simulink model "Shaddad_SensorModels"  (R2026b)
settings: Solver=VariableStepAuto
values from neighbouring files (symbols this model uses):
  D = zeros(nx, ny, 'uint8')    [sens_lidar2d_fast.m]
  P = (P + P.')/2    [sens_nav_ekf.m]
undefined symbols (not defined in the file or in its folder): sens_gnss_fixchain_prm, sens_lidar2d_fast_prm, Ts
libraries: sensorgpslib x3, uavsimlib x3, sharedutil x1
settings Model: Creator=aomar  LastModifiedBy=aomar

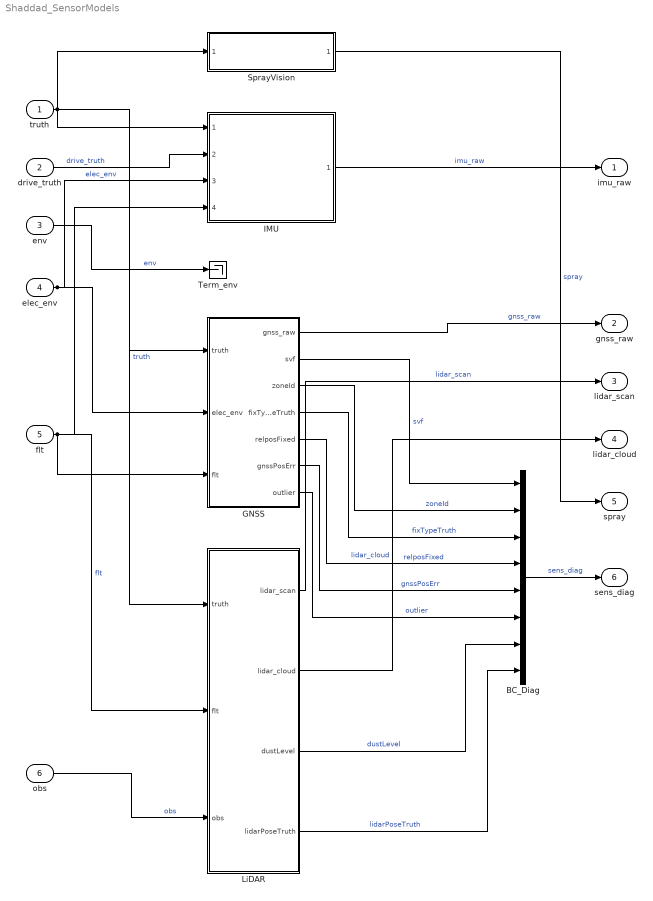
== system Shaddad_SensorModels ==
  truth : Inport  OutDataTypeStr=Bus: Bus_TruthState  SampleTime=Ts.base
  drive_truth : Inport  Port=2  OutDataTypeStr=Bus: Bus_DriveTruth  SampleTime=Ts.base
  env : Inport  Port=3  OutDataTypeStr=Bus: Bus_EnvState  SampleTime=Ts.hk
  elec_env : Inport  Port=4  OutDataTypeStr=Bus: Bus_ElecEnv  SampleTime=Ts.hk
  flt : Inport  Port=5  OutDataTypeStr=Bus: Bus_FaultInject  SampleTime=Ts.ctrl
  obs : Inport  Port=6  OutDataTypeStr=Bus: Bus_ObstaclesDyn  SampleTime=Ts.ctrl
  BC_Diag : BusCreator  Inputs=8  OutDataTypeStr=Bus: Bus_SensTruthDiag  NonVirtualBus=on
      settings: InheritFromInputs=off
  GNSS : Subsystem  Description=|
      | sens_gnss_model (T11, sensors spec 3.2). Ports: in 1 truth Bus_TruthState 0.001, 2 elec_env Bus_ElecEnv 0.1, 3 flt Bus_FaultInject 0.01; out 1 gnss_raw Bus_GnssRaw 0.1, 2 svf double, 3 zoneId uint8, 4 fixTypeTruth uint8, 5 relposFixed boolean, 6 gnssPosErr double[3] (reported - true antenna ENU), 7 outlier boolean (all 0.1).
      | p_a = pos_W + R_WB rAnt1, v_a = vel_W + R_WB (omega x rAnt1); Delay 8 x 0.01 s (latency) -> 0.1 s epochs; sky view = 2-D Lookup Tables P.world.gnssSvf (linear) / gnssZoneId (nearest) at the antenna xy (D59); fix chain MATLAB Function sens_gnss_fixchain (corrOK/corrAge from elec_env, gnss_outage / gnss_force_float from flt); three mspsensorlib/GPS (FIXED/FLOAT/SINGLE, position only: VelocityAccuracy 0) + Multiport Switch {4,5,1}; velocity v_a + N(0, sigVel(fix)^2) per axis (the GPS block's own velocity noise reads 1.2533 sigVel high along the track); outliers U(2,5) m; heading CW from N + N(0, 0.5 deg).
  IMU : Subsystem  ReferencedSubsystem=sens_imu_model
  LiDAR : Subsystem  Description=|
      | sens_lidar_model (T11, sensors spec 3.4). Ports: in 1 truth Bus_TruthState 0.001, 2 flt Bus_FaultInject 0.01, 3 obs Bus_ObstaclesDyn 0.01; out 1 lidar_scan Bus_LidarScanRaw 0.1, 2 lidar_cloud Bus_LidarCloudRaw 0.1, 3 dustLevel double 0.1, 4 lidarPoseTruth double[3] [x_E y_N psi] 0.1.
      | Variant Subsystem VC_LIDAR (update diagram): 1 FAST2D = MATLAB Function sens_lidar2d_fast (raster of P.world.obstacles at first call, film layer, dynamic obstacles from obs, dust, blackout), cloud = P.ic; 2 FULL3D = uavsimlib UAV Scenario Configuration (sens_uavScene from utilities/sens_env_to_uavscenario.m) / Motion Write / Lidar (interpreted only, short runs), scan = P.ic.
  SprayVision : Subsystem  ReferencedSubsystem=sens_spray_vision
  Term_env : Terminator
  imu_raw : Outport  OutDataTypeStr=Bus: Bus_ImuRaw
  gnss_raw : Outport  Port=2  OutDataTypeStr=Bus: Bus_GnssRaw
  lidar_scan : Outport  Port=3  OutDataTypeStr=Bus: Bus_LidarScanRaw
  lidar_cloud : Outport  Port=4  OutDataTypeStr=Bus: Bus_LidarCloudRaw
  spray : Outport  Port=5  OutDataTypeStr=Bus: Bus_SprayDemand
  sens_diag : Outport  Port=6  OutDataTypeStr=Bus: Bus_SensTruthDiag
  wires:
  truth/1 -> LiDAR/1(truth), GNSS/1(truth), SprayVision/1, IMU/1  "truth"
  drive_truth/1 -> IMU/2  "drive_truth"
  env/1 -> Term_env/1  "env"
  elec_env/1 -> GNSS/2(elec_env), IMU/3  "elec_env"
  flt/1 -> LiDAR/2(flt), IMU/4, GNSS/3(flt)  "flt"
  obs/1 -> LiDAR/3(obs)  "obs"
  GNSS/1(gnss_raw) -> gnss_raw/1  "gnss_raw"
  GNSS/2(svf) -> BC_Diag/1  "svf"
  GNSS/3(zoneId) -> BC_Diag/2  "zoneId"
  GNSS/4(fixTypeTruth) -> BC_Diag/3  "fixTypeTruth"
  GNSS/5(relposFixed) -> BC_Diag/4  "relposFixed"
  GNSS/7(outlier) -> BC_Diag/6  "outlier"
  LiDAR/2(lidar_cloud) -> lidar_cloud/1  "lidar_cloud"
  LiDAR/3(dustLevel) -> BC_Diag/7  "dustLevel"
  LiDAR/4(lidarPoseTruth) -> BC_Diag/8  "lidarPoseTruth"
  SprayVision/1 -> spray/1  "spray"
  IMU/1 -> imu_raw/1  "imu_raw"
  BC_Diag/1 -> sens_diag/1  "sens_diag"
  GNSS/6(gnssPosErr) -> BC_Diag/5  "gnssPosErr"
  LiDAR/1(lidar_scan) -> lidar_scan/1  "lidar_scan"

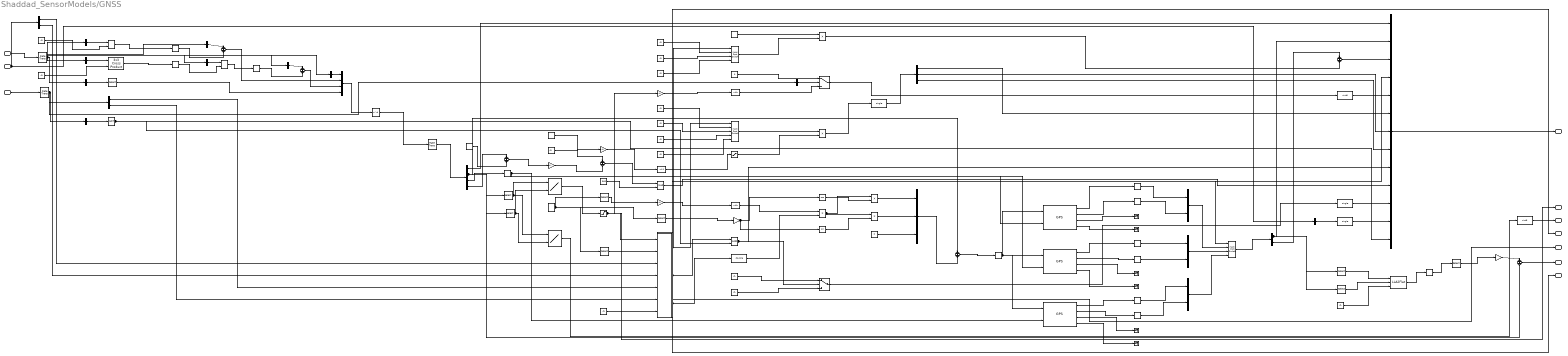
== system Shaddad_SensorModels/GNSS ==
  truth : Inport  OutDataTypeStr=Bus: Bus_TruthState  SampleTime=Ts.base
  elec_env : Inport  Port=2  OutDataTypeStr=Bus: Bus_ElecEnv  SampleTime=Ts.hk
  flt : Inport  Port=3  OutDataTypeStr=Bus: Bus_FaultInject  SampleTime=Ts.ctrl
  AccOut : Demux  Outputs=3
  AccRep : Product  Inputs=**
  AccSel : MultiPortSwitch  DataPortOrder=Specify indices  Inputs=4  DataPortIndices={4,5,1,0}  DiagnosticForDefault=None  SaturateOnIntegerOverflow=off  InputSameDT=off
  AccSingle : DataTypeConversion  OutDataTypeStr=single  RndMeth=Nearest  SaturateOnIntegerOverflow=off
  Acc_accFixed : Constant  Value=P.sensors.gnss.accFixed  SampleTime=Ts.gnss
  Acc_accFloat : Constant  Value=P.sensors.gnss.accFloat  SampleTime=Ts.gnss
  Acc_accNoFix : Constant  Value=P.sensors.gnss.accNoFix  SampleTime=Ts.gnss
  Acc_accSingle : Constant  Value=P.sensors.gnss.accSingle  SampleTime=Ts.gnss
  Alt : Selector  InputPortWidth=3  IndexOptions=Index vector (dialog)  Indices=3  OutputSizes=1
  AntX : Selector  InputPortWidth=3  IndexOptions=Index vector (dialog)  Indices=1  OutputSizes=1
  AntY : Selector  InputPortWidth=3  IndexOptions=Index vector (dialog)  Indices=2  OutputSizes=1
  BC_Gnss : BusCreator  Inputs=13  OutDataTypeStr=Bus: Bus_GnssRaw  NonVirtualBus=on
      settings: InheritFromInputs=off
  C360 : Constant  Value=360  SampleTime=Ts.gnss
  ChainPrm : Constant  Value=sens_gnss_fixchain_prm(P.sensors.gnss)
  Corr : BusSelector  OutputSignals=gnssCorrOK,gnssCorrAge
  CorrAgeS : DataTypeConversion  OutDataTypeStr=single  RndMeth=Nearest  SaturateOnIntegerOverflow=off
  Corr_gnssCorrAge : BusSelector  OutputSignals=gnssCorrAge
  CosDir : Trigonometry  Operator=cos
  Dir2Pi : Gain  Gain=2*pi
  Epoch : Demux  Outputs=[1 3 3 1]
  FixChain : MATLAB Function  TreatAsAtomicUnit=on
  FixSel : MultiPortSwitch  DataPortOrder=Specify indices  DataPortIndices={4,5,1}  DiagnosticForDefault=None  SaturateOnIntegerOverflow=off  InputSameDT=off
  Flt : BusSelector  OutputSignals=gnss_outage,gnss_force_float
  Flt_gnss_outage : BusSelector  OutputSignals=gnss_outage
  Flt_gnss_outage_2 : BusSelector  OutputSignals=gnss_outage
  GPS_FIXED : sensorgpslib/GPS  DispRefFrame=ENU  PositionInputFormat=Local  ReferenceLocation=P.sensors.refLLA  HorizontalPositionAccuracy=P.sensors.gnss.sigH(1)  VerticalPositionAccuracy=P.sensors.gnss.sigV(1)  VelocityAccuracy=0  DecayFactor=P.sensors.gnss.decay(1)  SeedDouble=P.sensors.gnss.seeds(1)  SimulateUsing=Code generation
      settings: LibrarySourceBlock=mspsensorlib/GPS
  GPS_FLOAT : sensorgpslib/GPS  DispRefFrame=ENU  PositionInputFormat=Local  ReferenceLocation=P.sensors.refLLA  HorizontalPositionAccuracy=P.sensors.gnss.sigH(2)  VerticalPositionAccuracy=P.sensors.gnss.sigV(2)  VelocityAccuracy=0  DecayFactor=P.sensors.gnss.decay(2)  SeedDouble=P.sensors.gnss.seeds(2)  SimulateUsing=Code generation
      settings: LibrarySourceBlock=mspsensorlib/GPS
  GPS_SINGLE : sensorgpslib/GPS  DispRefFrame=ENU  PositionInputFormat=Local  ReferenceLocation=P.sensors.refLLA  HorizontalPositionAccuracy=P.sensors.gnss.sigH(3)  VerticalPositionAccuracy=P.sensors.gnss.sigV(3)  VelocityAccuracy=0  DecayFactor=P.sensors.gnss.decay(3)  SeedDouble=P.sensors.gnss.seeds(3)  SimulateUsing=Code generation
      settings: LibrarySourceBlock=mspsensorlib/GPS
  GpsOut : Demux  Outputs=[3 3]
  Head90 : Constant  Value=90 - P.sensors.gnss.psiBaseline*180/pi  SampleTime=Ts.gnss
  HeadAcc : Switch  Criteria=u2 ~= 0  SaturateOnIntegerOverflow=off  InputSameDT=off
  HeadAccBad : Constant  Value=P.sensors.gnss.headAccInvalid_deg  SampleTime=Ts.gnss
  HeadAccOK : Constant  Value=P.sensors.gnss.head_sigma_deg  SampleTime=Ts.gnss
  HeadAccS : DataTypeConversion  OutDataTypeStr=single  RndMeth=Nearest  SaturateOnIntegerOverflow=off
  HeadCW : Sum  Inputs=+-
  HeadMod : Math  Operator=mod
  HeadNoise : RandomNumber  Variance=P.sensors.gnss.head_sigma^2  Seed=P.sensors.gnss.seedHead  SampleTime=Ts.gnss
  HeadValid : Logic  AllPortsSameDT=off  OutDataTypeStr=boolean
  Href : Constant  Value=-P.sensors.refLLA(3)  SampleTime=Ts.gnss
  Jump : Mux  Inputs=3
  JumpE : Product  Inputs=**
  JumpMag : Product  Inputs=**
  JumpN : Product  Inputs=**
  LLA1d_FIXED : Reshape
  LLA1d_FLOAT : Reshape
  LLA1d_SINGLE : Reshape
  LLA2Flat : LLA2Flat  LL0=P.sensors.refLLA(1:2)
  La_W : Reshape
  LatLon : Selector  InputPortWidth=3  IndexOptions=Index vector (dialog)  Indices=[1 2]  OutputSizes=1
  Latency : Delay  DelayLength=P.sensors.gnss.latencySteps  InitialCondition=0  SampleTime=Ts.ctrl
  MagMin : Bias  Bias=P.sensors.gnss.outlierMag(1)  SaturateOnIntegerOverflow=off
  MagSpan : Gain  Gain=P.sensors.gnss.outlierMag(2) - P.sensors.gnss.outlierMag(1)
  NED1d : Reshape
  NED2ENU : Gain  Gain=[1 1 -1]
  NED2ENU_sel : Selector  InputPortWidth=3  IndexOptions=Index vector (dialog)  Indices=[2 1 3]  OutputSizes=1
  NotOutage : Logic  Operator=NOT  Inputs=1  AllPortsSameDT=off  OutDataTypeStr=boolean
  OmegaXra : sharedutil/3x3 Cross Product  aMode=aMode
      settings: LibrarySourceBlock=aerolibutil/3x3 Cross Product
  Out_FIXED : Mux  Inputs=[3 3]
  Out_FLOAT : Mux  Inputs=[3 3]
  Out_SINGLE : Mux  Inputs=[3 3]
  OutlierD : DataTypeConversion  OutDataTypeStr=double  RndMeth=Nearest  SaturateOnIntegerOverflow=off
  PosAnt : Sum
  PosErr : Sum  Inputs=+-
  PosIn : Sum
  PosRow : Reshape  OutputDimensionality=Row vector (2-D)
  Psi : Selector  InputPortWidth=3  IndexOptions=Index vector (dialog)  Indices=1  OutputSizes=1
  PsiDeg : Gain  Gain=180/pi
  PsiMeas : Sum
  RT_epoch : RateTransition  OutPortSampleTime=Ts.gnss
  RT_flt : RateTransition  OutPortSampleTime=Ts.gnss
  RT_truth : RateTransition  OutPortSampleTime=Ts.ctrl
  RWB_ra : Product  Multiplication=Matrix(*)
  RWB_wxr : Product  Multiplication=Matrix(*)
  RepBias : Bias  Bias=1  SaturateOnIntegerOverflow=off
  RepClamp : Saturate  UpperLimit=P.sensors.gnss.repClamp(2)  LowerLimit=P.sensors.gnss.repClamp(1)
  RepGain : Gain  Gain=P.sensors.gnss.repJitter
  RepNoise : RandomNumber  Seed=P.sensors.gnss.seedJit  SampleTime=Ts.gnss
  SVF_Clamp : Saturate  UpperLimit=P.sensors.gnss.svfClamp(2)  LowerLimit=P.sensors.gnss.svfClamp(1)
  SVF_LUT : Lookup_n-D  BreakpointsForDimension1=P.world.terrain.xE  BreakpointsForDimension2=P.world.terrain.yN  IndexSearchMethod=Evenly spaced points  Table=P.world.gnssSvf  ExtrapMethod=Clip  InternalRulePriority=Speed  RndMeth=Simplest
      settings: InputPortMap=u0,u1
  SV_bias : Bias  Bias=P.sensors.gnss.numSV(1)  SaturateOnIntegerOverflow=off
  SV_gain : Gain  Gain=P.sensors.gnss.numSV(2)
  SV_out : Switch  Criteria=u2 ~= 0  SaturateOnIntegerOverflow=off  InputSameDT=off
  SV_u8 : DataTypeConversion  OutDataTypeStr=uint8  RndMeth=Nearest  SaturateOnIntegerOverflow=off
  SV_zero : Constant  Value=0  SampleTime=Ts.gnss
  SigVel_FIXED : Constant  Value=P.sensors.gnss.sigVel(1)  SampleTime=Ts.gnss
  SigVel_FLOAT : Constant  Value=P.sensors.gnss.sigVel(2)  SampleTime=Ts.gnss
  SigVel_SINGLE : Constant  Value=P.sensors.gnss.sigVel(3)  SampleTime=Ts.gnss
  SinDir : Trigonometry
  TermCrs_FIXED : Terminator
  TermCrs_FLOAT : Terminator
  TermCrs_SINGLE : Terminator
  TermGS_FIXED : Terminator
  TermGS_FLOAT : Terminator
  TermGS_SINGLE : Terminator
  TruthAnt : Mux  Inputs=[1 3 3 1]
  Truth_R_WB : BusSelector  OutputSignals=R_WB
  Truth_R_WB_2 : BusSelector  OutputSignals=R_WB
  Truth_eul : BusSelector  OutputSignals=eul
  Truth_omega_B : BusSelector  OutputSignals=omega_B
  Truth_pos_W : BusSelector  OutputSignals=pos_W
  Truth_t : BusSelector  OutputSignals=t
  Truth_vel_W : BusSelector  OutputSignals=vel_W
  U : UniformRandomNumber  Minimum=zeros(1,6)  Maximum=ones(1,6)  Seed=P.sensors.gnss.seedU  SampleTime=Ts.gnss
  U_chain : Selector  InputPortWidth=6  IndexOptions=Index vector (dialog)  Indices=1:4  OutputSizes=1
  U_dir : Selector  InputPortWidth=6  IndexOptions=Index vector (dialog)  Indices=6  OutputSizes=1
  U_mag : Selector  InputPortWidth=6  IndexOptions=Index vector (dialog)  Indices=5  OutputSizes=1
  Vel1d_FIXED : Reshape
  Vel1d_FLOAT : Reshape
  Vel1d_SINGLE : Reshape
  VelAnt : Sum
  VelMeas : Sum
  VelNoise : RandomNumber  Mean=[0 0 0]  Variance=[1 1 1]  Seed=P.sensors.gnss.seedVel  SampleTime=Ts.gnss
  VelNoiseS : Product  Inputs=**
  VelRow : Reshape  OutputDimensionality=Row vector (2-D)
  VelSigSel : MultiPortSwitch  DataPortOrder=Specify indices  DataPortIndices={4,5,1}  DiagnosticForDefault=None  SaturateOnIntegerOverflow=off  InputSameDT=off
  Wxr_W : Reshape
  Wxr_col : Reshape  OutputDimensionality=Column vector (2-D)
  Zero : Constant  Value=0  SampleTime=Ts.gnss
  ZoneU8 : DataTypeConversion  OutDataTypeStr=uint8  RndMeth=Nearest  SaturateOnIntegerOverflow=off
  Zone_LUT : Lookup_n-D  BreakpointsForDimension1=P.world.terrain.xE  BreakpointsForDimension2=P.world.terrain.yN  IndexSearchMethod=Evenly spaced points  Table=P.world.gnssZoneId  InterpMethod=Nearest  ExtrapMethod=Clip  InternalRulePriority=Speed  RndMeth=Simplest
      settings: InputPortMap=u0,u1
  r_a : Constant  Value=P.sensors.gnss.rAnt1
  r_a_col : Constant  Value=P.sensors.gnss.rAnt1(:)  VectorParams1D=off
  gnss_raw : Outport  OutDataTypeStr=Bus: Bus_GnssRaw
  svf : Outport  Port=2  OutDataTypeStr=double
  zoneId : Outport  Port=3  OutDataTypeStr=uint8
  fixTypeTruth : Outport  Port=4  OutDataTypeStr=uint8
  relposFixed : Outport  Port=5  OutDataTypeStr=boolean
  gnssPosErr : Outport  Port=6  OutDataTypeStr=double
  outlier : Outport  Port=7  OutDataTypeStr=boolean
  wires:
  truth/1 -> RT_truth/1  "truth"
  elec_env/1 -> Corr_gnssCorrAge/1, Corr/1  "elec_env"
  flt/1 -> RT_flt/1  "flt"
  Corr/1 -> FixChain/3(corrOK)  "<gnssCorrOK>"
  Corr/2 -> FixChain/4(corrAge)  "<gnssCorrAge>"
  r_a_col/1 -> RWB_ra/2  "r_a"
  r_a/1 -> OmegaXra/2  "r_a"
  RT_truth/1 -> Truth_eul/1, Truth_t/1, Truth_R_WB/1, Truth_pos_W/1, Truth_vel_W/1, Truth_R_WB_2/1, Truth_omega_B/1  "truth_10ms"
  RT_flt/1 -> Flt_gnss_outage_2/1, Flt/1, Flt_gnss_outage/1  "flt_100ms"
  Truth_R_WB/1 -> RWB_ra/1  "<R_WB>"
  Truth_omega_B/1 -> OmegaXra/1  "<omega_B>"
  Truth_eul/1 -> Psi/1  "<eul>"
  Flt_gnss_outage_2/1 -> NotOutage/1  "<gnss_outage>"
  Flt/1 -> FixChain/5(outage)  "<gnss_outage>"
  Flt/2 -> FixChain/6(forceFloat)  "<gnss_force_float>"
  RWB_ra/1 -> La_W/1  "RWB_ra"
  NotOutage/1 -> HeadValid/2, BC_Gnss/13  "newData"
  Psi/1 -> TruthAnt/4  "psi"
  OmegaXra/1 -> Wxr_col/1  "w_x_ra"
  La_W/1 -> PosAnt/2  "lever_W"
  Wxr_col/1 -> RWB_wxr/2  "Wxr_col"
  Truth_pos_W/1 -> PosAnt/1  "<pos_W>"
  Truth_R_WB_2/1 -> RWB_wxr/1  "<R_WB>"
  PosAnt/1 -> TruthAnt/2  "p_ant"
  RWB_wxr/1 -> Wxr_W/1  "RWB_wxr"
  Wxr_W/1 -> VelAnt/2  "w_x_ra_W"
  Truth_vel_W/1 -> VelAnt/1  "<vel_W>"
  VelAnt/1 -> TruthAnt/3  "v_ant"
  Truth_t/1 -> TruthAnt/1  "<t>"
  TruthAnt/1 -> Latency/1  "ant_truth"
  Latency/1 -> RT_epoch/1  "ant_truth_delayed"
  RT_epoch/1 -> Epoch/1  "ant_epoch"
  Epoch/1 -> BC_Gnss/1  "t_meas"
  Epoch/2 -> PosErr/2, PosIn/1, AntY/1, AntX/1  "p_ant_d"
  Epoch/3 -> VelRow/1  "v_ant_d"
  Epoch/4 -> PsiMeas/1  "psi_d"
  HeadNoise/1 -> PsiMeas/2  "n_head"
  PsiMeas/1 -> PsiDeg/1  "psi_meas"
  VelRow/1 -> GPS_SINGLE/2, GPS_FLOAT/2, GPS_FIXED/2  "VelRow"
  AntX/1 -> Zone_LUT/1, SVF_LUT/1  "x_ant"
  AntY/1 -> Zone_LUT/2, SVF_LUT/2  "y_ant"
  RepNoise/1 -> RepGain/1  "n_rep"
  Head90/1 -> HeadCW/1  "Head90"
  PsiDeg/1 -> HeadCW/2  "psi_deg"
  U/1 -> U_chain/1, U_dir/1, U_mag/1  "u"
  SVF_LUT/1 -> SVF_Clamp/1  "svf_raw"
  Zone_LUT/1 -> ZoneU8/1  "zone_dbl"
  HeadCW/1 -> HeadMod/1  "heading_unwrapped"
  RepGain/1 -> RepBias/1  "RepGain"
  C360/1 -> HeadMod/2  "C360"
  SVF_Clamp/1 -> SV_gain/1, FixChain/1(svf), svf/1  "svf"
  ChainPrm/1 -> FixChain/7(c)  "chain_prm"
  U_mag/1 -> MagSpan/1  "u_mag"
  U_chain/1 -> FixChain/2(u)  "u_chain"
  SigVel_FIXED/1 -> VelSigSel/2  "sigVel_FIXED"
  SigVel_FLOAT/1 -> VelSigSel/3  "sigVel_FLOAT"
  SigVel_SINGLE/1 -> VelSigSel/4  "sigVel_SINGLE"
  SV_gain/1 -> SV_bias/1  "SV_gain"
  Acc_accFixed/1 -> AccSel/2  "Acc_accFixed"
  Acc_accFloat/1 -> AccSel/3  "Acc_accFloat"
  Acc_accSingle/1 -> AccSel/4  "Acc_accSingle"
  Acc_accNoFix/1 -> AccSel/5  "Acc_accNoFix"
  HeadMod/1 -> BC_Gnss/10  "heading_deg"
  MagSpan/1 -> MagMin/1  "MagSpan"
  RepBias/1 -> RepClamp/1  "RepBias"
  U_dir/1 -> Dir2Pi/1  "u_dir"
  VelNoise/1 -> VelNoiseS/1  "n_vel"
  SV_zero/1 -> SV_out/1  "SV_zero"
  RepClamp/1 -> AccRep/2  "k_rep"
  HeadValid/1 -> BC_Gnss/9, HeadAcc/2  "headingValid"
  HeadAccOK/1 -> HeadAcc/1  "HeadAccOK"
  HeadAccBad/1 -> HeadAcc/3  "HeadAccBad"
  VelSigSel/1 -> VelNoiseS/2  "sig_vel"
  AccSel/1 -> AccRep/1  "acc_fix"
  SV_bias/1 -> SV_out/3  "numSV_dbl"
  MagMin/1 -> JumpMag/1  "jump"
  Dir2Pi/1 -> CosDir/1, SinDir/1  "dir"
  OutlierD/1 -> JumpMag/2  "outlier_d"
  Flt_gnss_outage/1 -> SV_out/2  "<gnss_outage>"
  VelNoiseS/1 -> VelMeas/2  "vel_noise"
  AccRep/1 -> AccSingle/1  "acc_rep"
  CosDir/1 -> JumpE/2  "CosDir"
  JumpMag/1 -> JumpE/1, JumpN/1  "jump_on"
  SinDir/1 -> JumpN/2  "SinDir"
  SV_out/1 -> SV_u8/1  "SV_out"
  HeadAcc/1 -> HeadAccS/1  "HeadAcc"
  JumpE/1 -> Jump/1  "JumpE"
  JumpN/1 -> Jump/2  "JumpN"
  Zero/1 -> Jump/3  "Zero"
  AccSingle/1 -> AccOut/1  "AccSingle"
  AccOut/1 -> BC_Gnss/6  "hAcc"
  AccOut/2 -> BC_Gnss/7  "vAcc"
  AccOut/3 -> BC_Gnss/8  "sAcc"
  Jump/1 -> PosIn/2  "jump_ENU"
  PosIn/1 -> PosRow/1  "p_in"
  PosRow/1 -> GPS_SINGLE/1, GPS_FIXED/1, GPS_FLOAT/1  "PosRow"
  GPS_FIXED/1 -> LLA1d_FIXED/1  "lla_FIXED"
  GPS_FIXED/2 -> Vel1d_FIXED/1  "vel_FIXED"
  GPS_FIXED/3 -> TermGS_FIXED/1  "groundspeed_FIXED"
  GPS_FIXED/4 -> TermCrs_FIXED/1  "course_FIXED"
  GPS_FLOAT/1 -> LLA1d_FLOAT/1  "lla_FLOAT"
  GPS_FLOAT/2 -> Vel1d_FLOAT/1  "vel_FLOAT"
  GPS_FLOAT/3 -> TermGS_FLOAT/1  "groundspeed_FLOAT"
  GPS_FLOAT/4 -> TermCrs_FLOAT/1  "course_FLOAT"
  GPS_SINGLE/1 -> LLA1d_SINGLE/1  "lla_SINGLE"
  GPS_SINGLE/2 -> Vel1d_SINGLE/1  "vel_SINGLE"
  GPS_SINGLE/3 -> TermGS_SINGLE/1  "groundspeed_SINGLE"
  GPS_SINGLE/4 -> TermCrs_SINGLE/1  "course_SINGLE"
  LLA1d_FIXED/1 -> Out_FIXED/1  "LLA1d_FIXED"
  Vel1d_FIXED/1 -> Out_FIXED/2  "Vel1d_FIXED"
  LLA1d_FLOAT/1 -> Out_FLOAT/1  "LLA1d_FLOAT"
  Vel1d_FLOAT/1 -> Out_FLOAT/2  "Vel1d_FLOAT"
  LLA1d_SINGLE/1 -> Out_SINGLE/1  "LLA1d_SINGLE"
  Vel1d_SINGLE/1 -> Out_SINGLE/2  "Vel1d_SINGLE"
  Out_FIXED/1 -> FixSel/2  "gps_FIXED"
  Out_FLOAT/1 -> FixSel/3  "gps_FLOAT"
  Out_SINGLE/1 -> FixSel/4  "gps_SINGLE"
  FixSel/1 -> GpsOut/1  "gps_sel"
  GpsOut/1 -> BC_Gnss/2, Alt/1, LatLon/1  "lla"
  GpsOut/2 -> VelMeas/1  "vel_gps"
  Corr_gnssCorrAge/1 -> CorrAgeS/1  "<gnssCorrAge>"
  VelMeas/1 -> BC_Gnss/3  "vel_ENU"
  Href/1 -> LLA2Flat/3  "href"
  LatLon/1 -> LLA2Flat/1  "latlon"
  Alt/1 -> LLA2Flat/2  "h"
  SV_u8/1 -> BC_Gnss/5  "numSV"
  HeadAccS/1 -> BC_Gnss/11  "headAcc_deg"
  CorrAgeS/1 -> BC_Gnss/12  "corrAge"
  BC_Gnss/1 -> gnss_raw/1  "gnss_raw"
  LLA2Flat/1 -> NED1d/1  "p_NED"
  NED1d/1 -> NED2ENU_sel/1  "NED1d"
  NED2ENU_sel/1 -> NED2ENU/1  "NED2ENU_sel"
  NED2ENU/1 -> PosErr/1  "p_rep_ENU"
  PosErr/1 -> gnssPosErr/1  "gnssPosErr"
  ZoneU8/1 -> zoneId/1  "zoneId"
  FixChain/1(fixType) -> VelSigSel/1, BC_Gnss/4, AccSel/1, fixTypeTruth/1, FixSel/1  "fixType"
  FixChain/2(relposFixed) -> HeadValid/1, relposFixed/1  "relposFixed"
  FixChain/3(outlier) -> OutlierD/1, outlier/1  "outlier"

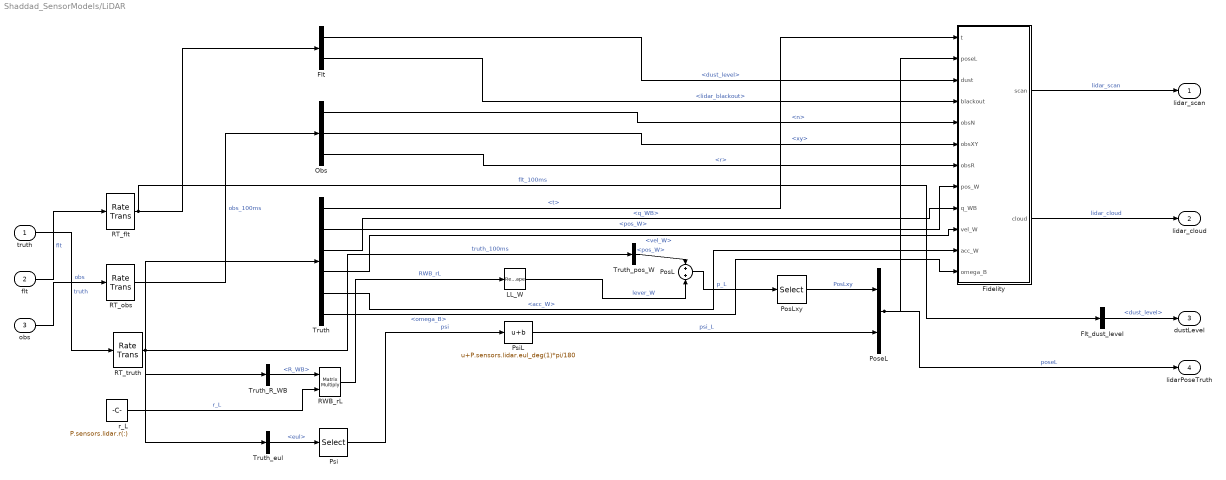
== system Shaddad_SensorModels/LiDAR ==
  truth : Inport  OutDataTypeStr=Bus: Bus_TruthState  SampleTime=Ts.base
  flt : Inport  Port=2  OutDataTypeStr=Bus: Bus_FaultInject  SampleTime=Ts.ctrl
  obs : Inport  Port=3  OutDataTypeStr=Bus: Bus_ObstaclesDyn  SampleTime=Ts.ctrl
  Fidelity : Subsystem  Variant=on
  Flt : BusSelector  OutputSignals=dust_level,lidar_blackout
  Flt_dust_level : BusSelector  OutputSignals=dust_level
  LL_W : Reshape
  Obs : BusSelector  OutputSignals=n,xy,r
  PosL : Sum
  PosLxy : Selector  InputPortWidth=3  IndexOptions=Index vector (dialog)  Indices=[1 2]  OutputSizes=1
  PoseL : Mux  Inputs=[2 1]
  Psi : Selector  InputPortWidth=3  IndexOptions=Index vector (dialog)  Indices=1  OutputSizes=1
  PsiL : Bias  Bias=P.sensors.lidar.eul_deg(1)*pi/180  SaturateOnIntegerOverflow=off
  RT_flt : RateTransition  OutPortSampleTime=Ts.lidar
  RT_obs : RateTransition  OutPortSampleTime=Ts.lidar
  RT_truth : RateTransition  OutPortSampleTime=Ts.lidar
  RWB_rL : Product  Multiplication=Matrix(*)
  Truth : BusSelector  OutputSignals=t,pos_W,q_WB,vel_W,acc_W,omega_B
  Truth_R_WB : BusSelector  OutputSignals=R_WB
  Truth_eul : BusSelector  OutputSignals=eul
  Truth_pos_W : BusSelector  OutputSignals=pos_W
  r_L : Constant  Value=P.sensors.lidar.r(:)  VectorParams1D=off
  lidar_scan : Outport  OutDataTypeStr=Bus: Bus_LidarScanRaw
  lidar_cloud : Outport  Port=2  OutDataTypeStr=Bus: Bus_LidarCloudRaw
  dustLevel : Outport  Port=3  OutDataTypeStr=double
  lidarPoseTruth : Outport  Port=4  OutDataTypeStr=double
  wires:
  truth/1 -> RT_truth/1  "truth"
  flt/1 -> RT_flt/1  "flt"
  obs/1 -> RT_obs/1  "obs"
  r_L/1 -> RWB_rL/2  "r_L"
  RT_flt/1 -> Flt/1, Flt_dust_level/1  "flt_100ms"
  RT_obs/1 -> Obs/1  "obs_100ms"
  RT_truth/1 -> Truth_pos_W/1, Truth_eul/1, Truth/1, Truth_R_WB/1  "truth_100ms"
  Truth_R_WB/1 -> RWB_rL/1  "<R_WB>"
  Truth_eul/1 -> Psi/1  "<eul>"
  Flt/1 -> Fidelity/3(dust)  "<dust_level>"
  Flt/2 -> Fidelity/4(blackout)  "<lidar_blackout>"
  Obs/1 -> Fidelity/5(obsN)  "<n>"
  Obs/2 -> Fidelity/6(obsXY)  "<xy>"
  Obs/3 -> Fidelity/7(obsR)  "<r>"
  Truth/1 -> Fidelity/1(t)  "<t>"
  Truth/2 -> Fidelity/8(pos_W)  "<pos_W>"
  Truth/3 -> Fidelity/9(q_WB)  "<q_WB>"
  Truth/4 -> Fidelity/10(vel_W)  "<vel_W>"
  Truth/5 -> Fidelity/11(acc_W)  "<acc_W>"
  Truth/6 -> Fidelity/12(omega_B)  "<omega_B>"
  RWB_rL/1 -> LL_W/1  "RWB_rL"
  Psi/1 -> PsiL/1  "psi"
  LL_W/1 -> PosL/2  "lever_W"
  PsiL/1 -> PoseL/2  "psi_L"
  Truth_pos_W/1 -> PosL/1  "<pos_W>"
  PosL/1 -> PosLxy/1  "p_L"
  PosLxy/1 -> PoseL/1  "PosLxy"
  PoseL/1 -> Fidelity/2(poseL), lidarPoseTruth/1  "poseL"
  Fidelity/1(scan) -> lidar_scan/1  "lidar_scan"
  Fidelity/2(cloud) -> lidar_cloud/1  "lidar_cloud"
  Flt_dust_level/1 -> dustLevel/1  "<dust_level>"

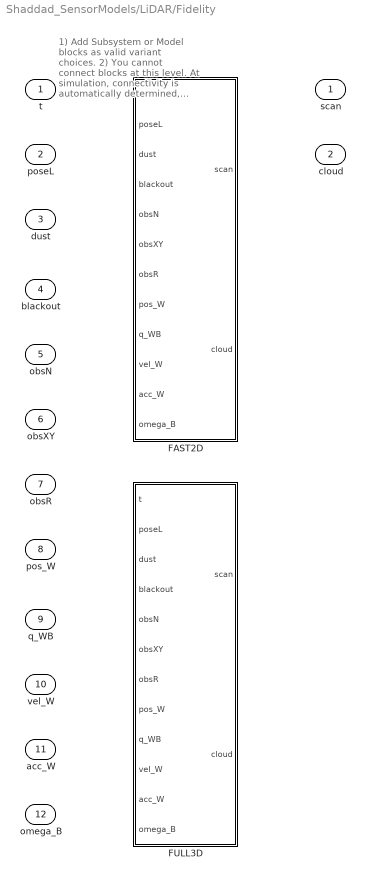
== system Shaddad_SensorModels/LiDAR/Fidelity ==
  note: 1) Add Subsystem or Model blocks as valid variant choices.
      | 2) You cannot connect blocks at this level. At simulation, connectivity is automatically
      | determined, based on the active variant and port name matching.
  t : Inport
  poseL : Inport  Port=2
  dust : Inport  Port=3
  blackout : Inport  Port=4
  obsN : Inport  Port=5
  obsXY : Inport  Port=6
  obsR : Inport  Port=7
  pos_W : Inport  Port=8
  q_WB : Inport  Port=9
  vel_W : Inport  Port=10
  acc_W : Inport  Port=11
  omega_B : Inport  Port=12
  FAST2D : Subsystem  Description=FAST2D (VC_LIDAR == 1): 360-beam height-band scan, lidar_cloud = P.ic.Bus_LidarCloudRaw.  VariantControl=VC_LIDAR == 1
  FULL3D : Subsystem  Description=FULL3D (VC_LIDAR == 2): uavScenario sens_uavScene (base), platform Shaddad with sensor Lidar; organised cloud padded with NaN to [32 1024 3]; lidar_scan = P.ic.Bus_LidarScanRaw. Interpreted only.  VariantControl=VC_LIDAR == 2
  scan : Outport
  cloud : Outport  Port=2

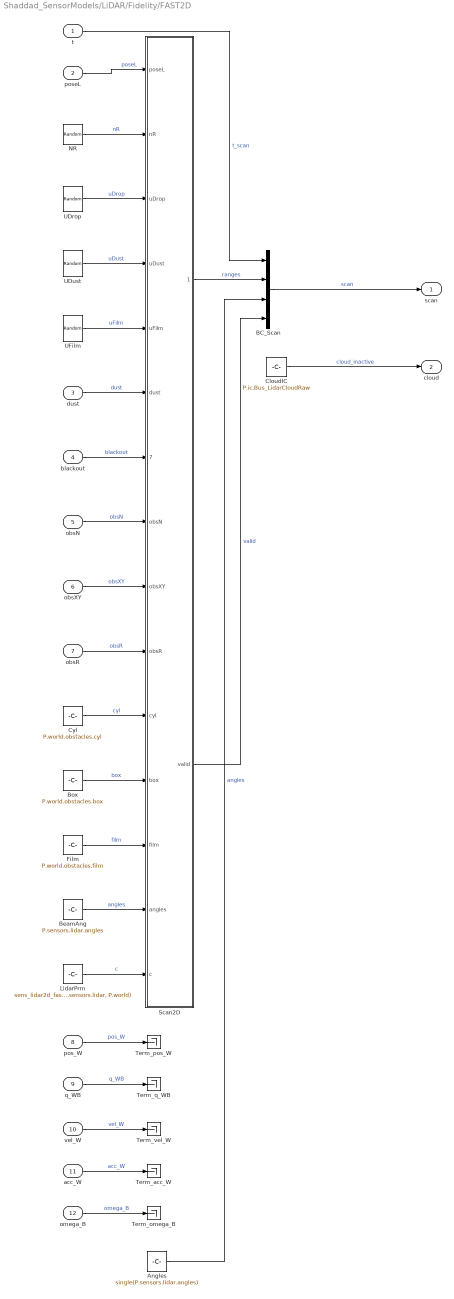
== system Shaddad_SensorModels/LiDAR/Fidelity/FAST2D ==
  t : Inport
  poseL : Inport  Port=2
  dust : Inport  Port=3
  blackout : Inport  Port=4
  obsN : Inport  Port=5
  obsXY : Inport  Port=6
  obsR : Inport  Port=7
  pos_W : Inport  Port=8
  q_WB : Inport  Port=9
  vel_W : Inport  Port=10
  acc_W : Inport  Port=11
  omega_B : Inport  Port=12
  Angles : Constant  Value=single(P.sensors.lidar.angles)  OutDataTypeStr=single  SampleTime=Ts.lidar
  BC_Scan : BusCreator  Inputs=4  OutDataTypeStr=Bus: Bus_LidarScanRaw  NonVirtualBus=on
      settings: InheritFromInputs=off
  BeamAng : Constant  Value=P.sensors.lidar.angles  VectorParams1D=off
  Box : Constant  Value=P.world.obstacles.box  VectorParams1D=off
  CloudIC : Constant  Value=P.ic.Bus_LidarCloudRaw  OutDataTypeStr=Bus: Bus_LidarCloudRaw  SampleTime=Ts.lidar
  Cyl : Constant  Value=P.world.obstacles.cyl  VectorParams1D=off
  Film : Constant  Value=P.world.obstacles.film  VectorParams1D=off
  LidarPrm : Constant  Value=sens_lidar2d_fast_prm(P.sensors.lidar, P.world)  VectorParams1D=off
  NR : RandomNumber  Mean=zeros(1,P.sensors.lidar.nBeams)  Variance=ones(1,P.sensors.lidar.nBeams)  Seed=P.sensors.lidar.seedNR  SampleTime=Ts.lidar
  Scan2D : MATLAB Function  TreatAsAtomicUnit=on
  Term_acc_W : Terminator
  Term_omega_B : Terminator
  Term_pos_W : Terminator
  Term_q_WB : Terminator
  Term_vel_W : Terminator
  UDrop : UniformRandomNumber  Minimum=zeros(1,P.sensors.lidar.nBeams)  Maximum=ones(1,P.sensors.lidar.nBeams)  Seed=P.sensors.lidar.seedDrop  SampleTime=Ts.lidar
  UDust : UniformRandomNumber  Minimum=zeros(1,P.sensors.lidar.nBeams)  Maximum=ones(1,P.sensors.lidar.nBeams)  Seed=P.sensors.lidar.seedDust  SampleTime=Ts.lidar
  UFilm : UniformRandomNumber  Minimum=zeros(1,P.sensors.lidar.nBeams)  Maximum=ones(1,P.sensors.lidar.nBeams)  Seed=P.sensors.lidar.seedFilm  SampleTime=Ts.lidar
  scan : Outport
  cloud : Outport  Port=2
  wires:
  t/1 -> BC_Scan/1  "t_scan"
  poseL/1 -> Scan2D/1(poseL)  "poseL"
  NR/1 -> Scan2D/2(nR)  "nR"
  UDrop/1 -> Scan2D/3(uDrop)  "uDrop"
  UDust/1 -> Scan2D/4(uDust)  "uDust"
  UFilm/1 -> Scan2D/5(uFilm)  "uFilm"
  dust/1 -> Scan2D/6(dust)  "dust"
  blackout/1 -> Scan2D/7(blackout)  "blackout"
  obsN/1 -> Scan2D/8(obsN)  "obsN"
  obsXY/1 -> Scan2D/9(obsXY)  "obsXY"
  obsR/1 -> Scan2D/10(obsR)  "obsR"
  Cyl/1 -> Scan2D/11(cyl)  "cyl"
  Box/1 -> Scan2D/12(box)  "box"
  Film/1 -> Scan2D/13(film)  "film"
  BeamAng/1 -> Scan2D/14(angles)  "angles"
  LidarPrm/1 -> Scan2D/15(c)  "c"
  pos_W/1 -> Term_pos_W/1  "pos_W"
  q_WB/1 -> Term_q_WB/1  "q_WB"
  vel_W/1 -> Term_vel_W/1  "vel_W"
  acc_W/1 -> Term_acc_W/1  "acc_W"
  omega_B/1 -> Term_omega_B/1  "omega_B"
  Angles/1 -> BC_Scan/3  "angles"
  Scan2D/1(ranges) -> BC_Scan/2  "ranges"
  Scan2D/2(valid) -> BC_Scan/4  "valid"
  BC_Scan/1 -> scan/1  "scan"
  CloudIC/1 -> cloud/1  "cloud_inactive"

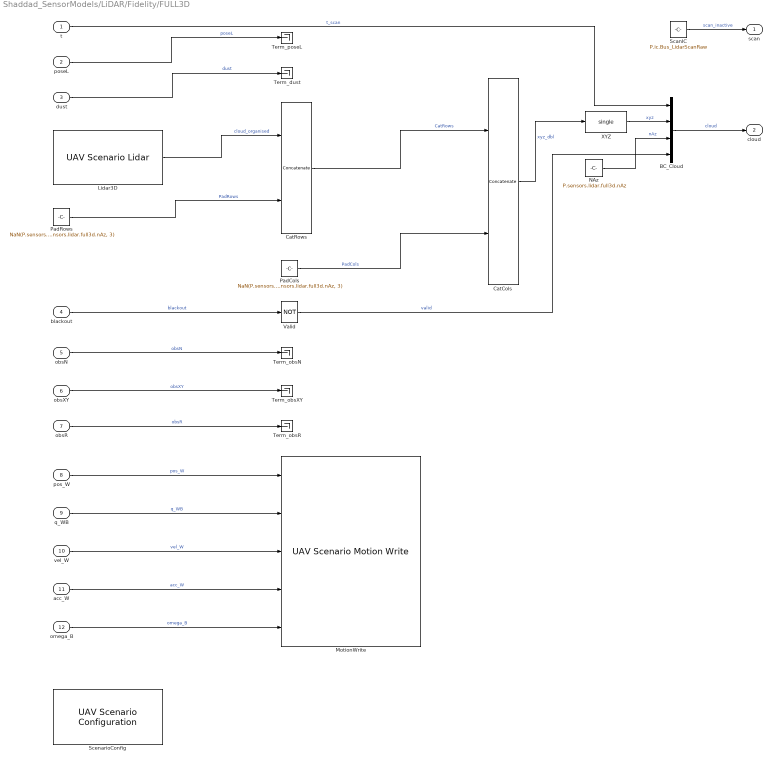
== system Shaddad_SensorModels/LiDAR/Fidelity/FULL3D ==
  t : Inport
  poseL : Inport  Port=2
  dust : Inport  Port=3
  blackout : Inport  Port=4
  obsN : Inport  Port=5
  obsXY : Inport  Port=6
  obsR : Inport  Port=7
  pos_W : Inport  Port=8
  q_WB : Inport  Port=9
  vel_W : Inport  Port=10
  acc_W : Inport  Port=11
  omega_B : Inport  Port=12
  BC_Cloud : BusCreator  Inputs=4  OutDataTypeStr=Bus: Bus_LidarCloudRaw  NonVirtualBus=on
      settings: InheritFromInputs=off
  CatCols : Concatenate  Mode=Multidimensional array  ConcatenateDimension=2
  CatRows : Concatenate  Mode=Multidimensional array
  Lidar3D : uavsimlib/UAV Scenario Lidar  Priority=1  SensorName=Shaddad/Lidar  MaxRange=P.sensors.lidar.full3d.MaxRange  RangeAccuracy=P.sensors.lidar.full3d.RangeAccuracy  AzimuthLimits=P.sensors.lidar.full3d.AzimuthLimits  AzimuthResolution=P.sensors.lidar.full3d.AzimuthResolution  ElevationLimits=P.sensors.lidar.full3d.ElevationLimits  ElevationResolution=P.sensors.lidar.full3d.ElevationResolution  HasNoise=on  HasOrganizedOutput=on  SampleTime=Ts.lidar
  MotionWrite : uavsimlib/UAV Scenario Motion Write  Priority=0  PlatName='Shaddad'  ReferenceFrame=ENU
  NAz : Constant  Value=P.sensors.lidar.full3d.nAz  OutDataTypeStr=uint16  SampleTime=Ts.lidar
  PadCols : Constant  Value=NaN(P.sensors.lidar.cloudSize(1), P.sensors.lidar.cloudSize(2) - P.sensors.lidar.full3d.nAz, 3)  SampleTime=Ts.lidar
  PadRows : Constant  Value=NaN(P.sensors.lidar.cloudSize(1) - P.sensors.lidar.full3d.nEl, P.sensors.lidar.full3d.nAz, 3)  SampleTime=Ts.lidar
  ScanIC : Constant  Value=P.ic.Bus_LidarScanRaw  OutDataTypeStr=Bus: Bus_LidarScanRaw  SampleTime=Ts.lidar
  ScenarioConfig : uavsimlib/UAV Scenario Configuration  Priority=-1  UAVScenarioObject=sens_uavScene  SampleTime=Ts.lidar  UpdateParam=false  SensorMotionBusName='SensorMotionBus'  PlatformMotionBusName='PlatformMotionBus'  ScenarioMotionBusName='ScenarioMotionBus'  ScenarioMotionSignalName='ScenarioMotions'
  Term_dust : Terminator
  Term_obsN : Terminator
  Term_obsR : Terminator
  Term_obsXY : Terminator
  Term_poseL : Terminator
  Valid : Logic  Operator=NOT  Inputs=1  AllPortsSameDT=off  OutDataTypeStr=boolean
  XYZ : DataTypeConversion  OutDataTypeStr=single  RndMeth=Nearest  SaturateOnIntegerOverflow=off
  scan : Outport
  cloud : Outport  Port=2
  wires:
  t/1 -> BC_Cloud/1  "t_scan"
  poseL/1 -> Term_poseL/1  "poseL"
  dust/1 -> Term_dust/1  "dust"
  PadRows/1 -> CatRows/2  "PadRows"
  blackout/1 -> Valid/1  "blackout"
  obsN/1 -> Term_obsN/1  "obsN"
  obsXY/1 -> Term_obsXY/1  "obsXY"
  obsR/1 -> Term_obsR/1  "obsR"
  pos_W/1 -> MotionWrite/1  "pos_W"
  q_WB/1 -> MotionWrite/2  "q_WB"
  vel_W/1 -> MotionWrite/3  "vel_W"
  acc_W/1 -> MotionWrite/4  "acc_W"
  omega_B/1 -> MotionWrite/5  "omega_B"
  Lidar3D/1 -> CatRows/1  "cloud_organised"
  PadCols/1 -> CatCols/2  "PadCols"
  Valid/1 -> BC_Cloud/4  "valid"
  CatRows/1 -> CatCols/1  "CatRows"
  CatCols/1 -> XYZ/1  "xyz_dbl"
  NAz/1 -> BC_Cloud/3  "nAz"
  XYZ/1 -> BC_Cloud/2  "xyz"
  BC_Cloud/1 -> cloud/1  "cloud"
  ScanIC/1 -> scan/1  "scan_inactive"

== matlab function Shaddad_SensorModels/LiDAR/Fidelity/FAST2D/Scan2D ==
  settings: description=FAST2D height-band ray casting (sensors spec 3.4, F3): subsystems/sensors/sens_lidar2d_fast.m; constants on inputs 11..15 (P.world.obstacles.cyl/box/film, P.sensors.lidar.angles, sens_lidar2d_fast_prm(P.sensors.lidar, P.world))
  data: poseL input; ranges output; nR input; uDrop input; uDust input; uFilm input; dust input; blackout input; obsN input; obsXY input; obsR input; cyl input; box input; film input; angles input; c input; valid output
function [ranges, valid] = fcn(poseL, nR, uDrop, uDust, uFilm, dust, blackout, obsN, obsXY, obsR, cyl, box, film, angles, c)
%#codegen
[ranges, valid] = sens_lidar2d_fast(poseL, nR, uDrop, uDust, uFilm, dust, blackout, obsN, obsXY, obsR, cyl, box, film, angles, c);

== matlab function Shaddad_SensorModels/GNSS/FixChain ==
  settings: description=RTK fix-state Markov chain (sensors spec 3.2, F2): subsystems/sensors/sens_gnss_fixchain.m; input c = sens_gnss_fixchain_prm(P.sensors.gnss)
  data: svf input; u input; fixType output; corrOK input; corrAge input; outage input; forceFloat input; c input; relposFixed output; outlier output
function [fixType, relposFixed, outlier] = fcn(svf, u, corrOK, corrAge, outage, forceFloat, c)
%#codegen
[fixType, relposFixed, outlier] = sens_gnss_fixchain(svf, u, corrOK, corrAge, outage, forceFloat, c);
